simulink model "sim2"  (R2025a)
settings: Solver=VariableStepAuto  StartTime=0.0  StopTime=10.0  RelTol=1e-3
values from neighbouring files (symbols this model uses):
  D = 0.25    [lw6.m]
  i_p = n_nom/n_rpm    (= 14.0622222222)    [lw6.m]
  J_gv = ro_gv*pi*(D/2)^4*h/2    (= 0.0118116520667)    [lw6.m]
  J_sum = 35.9e-7    (= 3.59e-06)    [lw6.m]
  k1 = 0.194    [lw6.m]
  k2 = 0.032    [lw6.m]
  k_m = 19.9e-3    (= 0.0199)    [lw6.m]
  L_a = 0.070e-3    (= 7e-05)    [lw6.m]
  Lxb = 0.19    [lw7.m]
  Lym = 0.31    [lw7.m]
  Lzb = 0.21    [lw7.m]
  R_a = 0.358    [lw6.m]
  ro = 1000    [lw6.m]
  Sat_low = -20    [lw7.m]
  Sat_up = 20    [lw7.m]
  U_nom = 18    [lw6.m]
  w_0 = n_0 * 2 * pi / 60    (= 899.542696478)    [lw6.m]
settings Model: Creator=user  LastModifiedBy=user

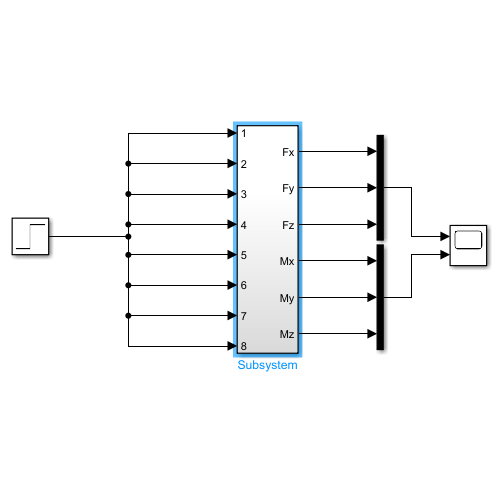
[thumbnail: Simulink's stored preview of the top-level diagram]
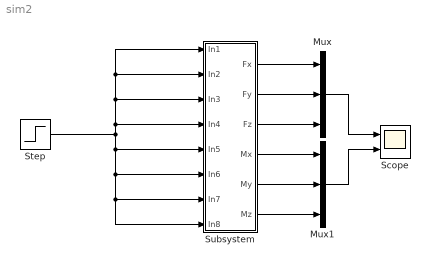
== system sim2 ==
  Mux : Mux  Inputs=3
  Mux1 : Mux  Inputs=3
  Scope : Scope  NumInputPorts=2
  Step : Step  SampleTime=0
  Subsystem : Subsystem
  wires:
  Step/1 -> Subsystem/7(In7), Subsystem/8(In8), Subsystem/6(In6), Subsystem/5(In5), Subsystem/3(In3), Subsystem/2(In2), Subsystem/1(In1), Subsystem/4(In4)
  Subsystem/1(Fx) -> Mux/1
  Subsystem/2(Fy) -> Mux/2
  Subsystem/3(Fz) -> Mux/3
  Subsystem/4(Mx) -> Mux1/1
  Subsystem/5(My) -> Mux1/2
  Subsystem/6(Mz) -> Mux1/3
  Mux/1 -> Scope/1
  Mux1/1 -> Scope/2

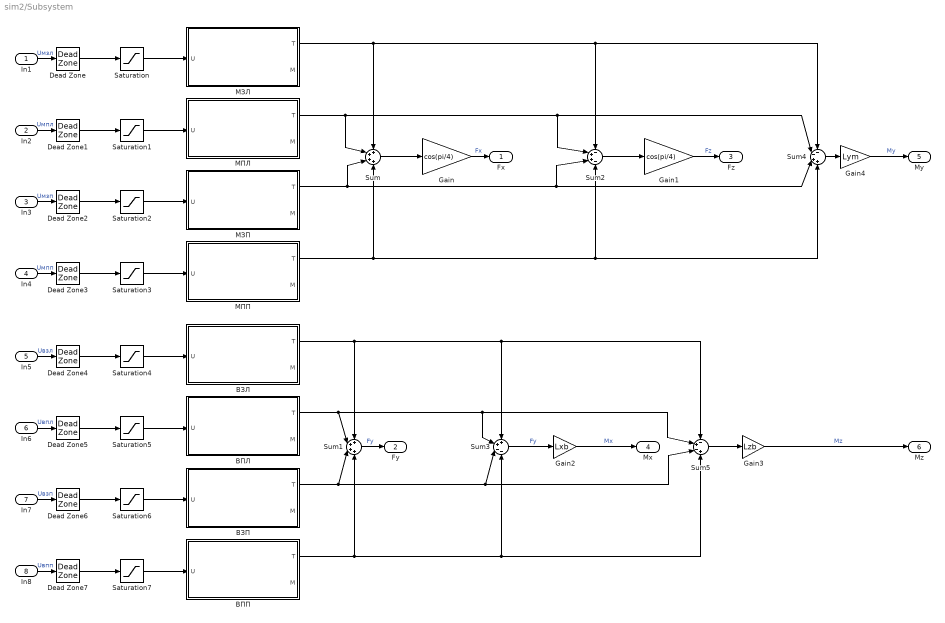
== system sim2/Subsystem ==
  In1 : Inport
  In2 : Inport  Port=2
  In3 : Inport  Port=3
  In4 : Inport  Port=4
  In5 : Inport  Port=5
  In6 : Inport  Port=6
  In7 : Inport  Port=7
  In8 : Inport  Port=8
  Dead Zone{,1..7} (8 alike) : DeadZone  LowerValue=Dead_low  UpperValue=Dead_up
  Gain : Gain  Gain=cos(pi/4)
  Gain1 : Gain  Gain=cos(pi/4)
  Gain2 : Gain  Gain=Lxb
  Gain3 : Gain  Gain=Lzb
  Gain4 : Gain  Gain=Lym
  Saturation{,1..7} (8 alike) : Saturate  UpperLimit=Sat_up  LowerLimit=Sat_low
  Sum : Sum  Inputs=++++
  Sum1 : Sum  Inputs=++++
  Sum2 : Sum  Inputs=-++-
  Sum3 : Sum  Inputs=++--
  Sum4 : Sum  Inputs=--++
  Sum5 : Sum  Inputs=-+-+
  ВЗЛ : Subsystem
  ВЗП : Subsystem
  ВПЛ : Subsystem
  ВПП : Subsystem
  МЗЛ : Subsystem
  МЗП : Subsystem
  МПЛ : Subsystem
  МПП : Subsystem
  Fx : Outport
  Fy : Outport  Port=2
  Fz : Outport  Port=3
  Mx : Outport  Port=4
  My : Outport  Port=5
  Mz : Outport  Port=6
  wires:
  In5/1 -> Dead Zone4/1  "Uвзл"
  Sum4/1 -> Gain4/1
  Gain1/1 -> Fz/1  "Fz"
  Sum5/1 -> Gain3/1
  In6/1 -> Dead Zone5/1  "Uвпл"
  Gain/1 -> Fx/1  "Fx"
  Sum/1 -> Gain/1
  Sum1/1 -> Fy/1  "Fy"
  Gain4/1 -> My/1  "My"
  ВЗП/1(T) -> Sum5/3, Sum3/3, Sum1/3
  In4/1 -> Dead Zone3/1  "Uмпп"
  Sum3/1 -> Gain2/1  "Fy"
  In8/1 -> Dead Zone7/1  "Uвпп"
  Sum2/1 -> Gain1/1
  МЗЛ/1(T) -> Sum4/1, Sum2/1, Sum/1
  ВПЛ/1(T) -> Sum5/2, Sum3/2, Sum1/2
  In2/1 -> Dead Zone1/1  "Uмпл"
  In1/1 -> Dead Zone/1  "Uмзл"
  In7/1 -> Dead Zone6/1  "Uвзп"
  Dead Zone3/1 -> Saturation3/1
  МЗП/1(T) -> Sum4/3, Sum2/3, Sum/3
  МПЛ/1(T) -> Sum4/2, Sum2/2, Sum/2
  МПП/1(T) -> Sum4/4, Sum2/4, Sum/4
  Saturation7/1 -> ВПП/1(U)
  Saturation3/1 -> МПП/1(U)
  Saturation6/1 -> ВЗП/1(U)
  Saturation2/1 -> МЗП/1(U)
  Dead Zone1/1 -> Saturation1/1
  Dead Zone2/1 -> Saturation2/1
  In3/1 -> Dead Zone2/1  "Uмзп"
  ВПП/1(T) -> Sum5/4, Sum3/4, Sum1/4
  Saturation/1 -> МЗЛ/1(U)
  Gain3/1 -> Mz/1  "Mz"
  Saturation5/1 -> ВПЛ/1(U)
  ВЗЛ/1(T) -> Sum5/1, Sum3/1, Sum1/1
  Dead Zone7/1 -> Saturation7/1
  Dead Zone4/1 -> Saturation4/1
  Gain2/1 -> Mx/1  "Mx"
  Dead Zone5/1 -> Saturation5/1
  Dead Zone/1 -> Saturation/1
  Dead Zone6/1 -> Saturation6/1
  Saturation4/1 -> ВЗЛ/1(U)
  Saturation1/1 -> МПЛ/1(U)

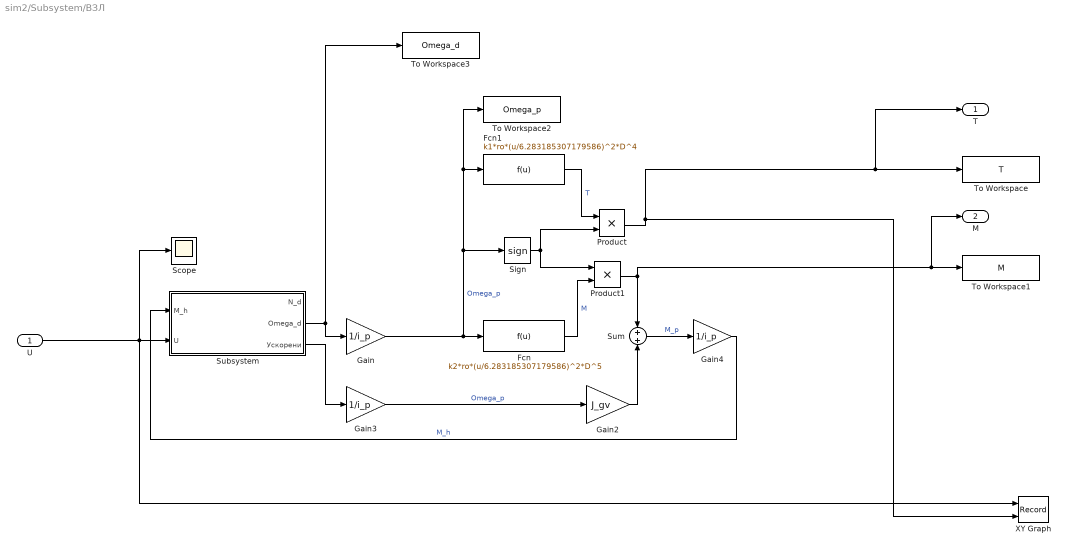
== system sim2/Subsystem/ВЗЛ ==
  U : Inport
  Fcn : Fcn  Expr=k2*ro*(u/6.283185307179586)^2*D^5
  Fcn1 : Fcn  Expr=k1*ro*(u/6.283185307179586)^2*D^4
  Gain : Gain  Gain=1/i_p
  Gain2 : Gain  Gain=J_gv
  Gain3 : Gain  Gain=1/i_p
  Gain4 : Gain  Gain=1/i_p
  Product : Product
  Product1 : Product
  Scope : Scope
      settings: ActiveDisplayYMinimum=-1  ActiveDisplayYMaximum=1
  Sign : Signum
  Subsystem : Subsystem
  Sum : Sum
  To Workspace : ToWorkspace  VariableName=T  SaveFormat=Timeseries  SampleTime=-1
  To Workspace1 : ToWorkspace  VariableName=M  SaveFormat=Timeseries  SampleTime=-1
  To Workspace2 : ToWorkspace  VariableName=Omega_p  SaveFormat=Timeseries  SampleTime=-1
  To Workspace3 : ToWorkspace  VariableName=Omega_d  SaveFormat=Timeseries  SampleTime=-1
  XY Graph : Record  NumPorts=2.0  FileSettingsInternal="{\"entries\":[{\"content\":{\"excelSettings\":{\"content\":{},\"type\":\"Streamout.ExcelSettings\"},\"parquetSettings\":{\"content\":{},\"type\":\"Streamout.ParquetSettings\"}},\"type\":\"Streamout.FileSettingStorage\",\"uuid\":\"\"}],\"packageUris\":[\"http:\\/\\/schema.mathworks.com\\/mf0\\/streamout_blocks\\/R2020a\"],\"version\":\"1.0\"}"  FrameSettings=[0, 0]  Layout=[1 1]  SignalsInternal="{\"entries\":[{\"content\":{\"signals\":[{\"content\":{\"blockPath\":[],\"dimensions\":[1],\"domain\":\"\",\"lineColor\":\"#a2142f\",\"plots\":[ 1 ],\"port\":1,\"signalID\":1,\"signalName\":\"Manual Switch\"},\"type\":\"RecordBlkView.Signal\",\"uuid\":\"\"},{\"content\":{\"blockPath\":[],\"dimensions\":[1],\"domain\":\"\",\"lineColor\":\"#139fff\",\"plots\":[ 1 ],\"port\":2,\"signalID\":2,\"signalName\":\"Product\"},\"type\":\"RecordBlkView.Signal\",\"uuid\":\"\"}]},\"type\":\"RecordBlkView.InputSignals\",\"uuid\":\"\"}],\"packageUris\":[\"http:\\/\\/schema.mathworks.com\\/mf0\\/streamout_blocks\\/R2020a\"],\"version\":\"1.0\"}"  VisualizationBindings="{\"xyplotplugin\":{\"info\":[{\"series\":[{\"bindingParametersList\":[{\"parameter\":\"X-Axis\",\"signalID\":1,\"signalName\":\"Manual Switch\"},{\"parameter\":\"Y-Axis\",\"signalID\":2,\"signalName\":\"Product\"}],\"seriesID\":0}],\"subplotID\":1}]}}"  CompatibilityTag=XY
  T : Outport
  M : Outport  Port=2
  wires:
  Gain3/1 -> Gain2/1  "Omega_p"
  Subsystem/3(Ускорени) -> Gain3/1
  Fcn1/1 -> Product/1  "T"
  Subsystem/2(Omega_d) -> Gain/1, To Workspace3/1
  Gain/1 -> Fcn/1, To Workspace2/1, Fcn1/1, Sign/1  "Omega_p"
  Sum/1 -> Gain4/1  "M_p"
  Sign/1 -> Product/2, Product1/1
  Product/1 -> T/1, To Workspace/1, XY Graph/2
  Gain4/1 -> Subsystem/1(M_h)  "M_h"
  Product1/1 -> Sum/1, M/1, To Workspace1/1
  U/1 -> Scope/1, XY Graph/1, Subsystem/2(U)
  Fcn/1 -> Product1/2  "M"
  Gain2/1 -> Sum/2

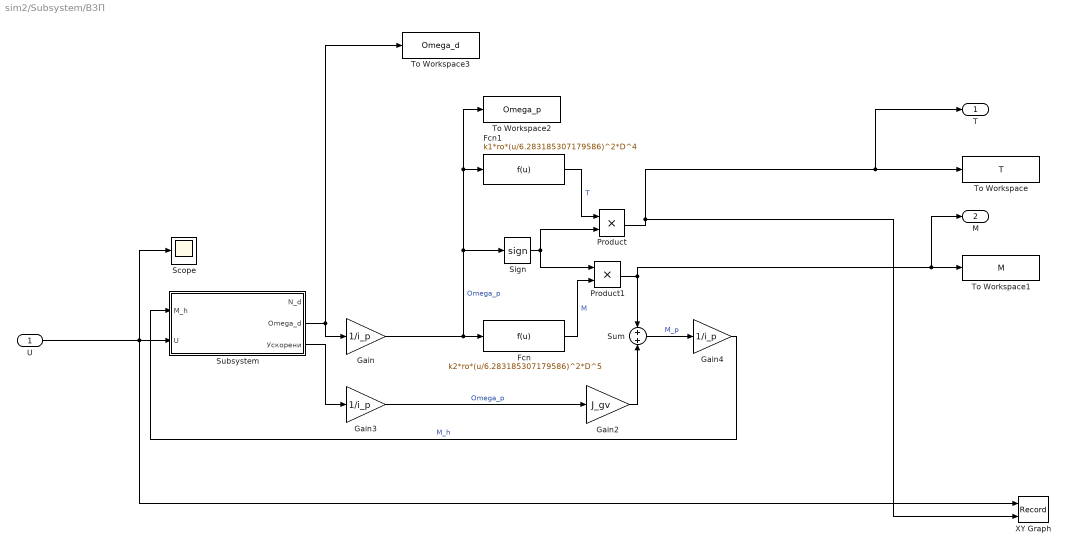
== system sim2/Subsystem/ВЗП ==
  U : Inport
  Fcn : Fcn  Expr=k2*ro*(u/6.283185307179586)^2*D^5
  Fcn1 : Fcn  Expr=k1*ro*(u/6.283185307179586)^2*D^4
  Gain : Gain  Gain=1/i_p
  Gain2 : Gain  Gain=J_gv
  Gain3 : Gain  Gain=1/i_p
  Gain4 : Gain  Gain=1/i_p
  Product : Product
  Product1 : Product
  Scope : Scope
      settings: ActiveDisplayYMinimum=-1  ActiveDisplayYMaximum=1
  Sign : Signum
  Subsystem : Subsystem
  Sum : Sum
  To Workspace : ToWorkspace  VariableName=T  SaveFormat=Timeseries  SampleTime=-1
  To Workspace1 : ToWorkspace  VariableName=M  SaveFormat=Timeseries  SampleTime=-1
  To Workspace2 : ToWorkspace  VariableName=Omega_p  SaveFormat=Timeseries  SampleTime=-1
  To Workspace3 : ToWorkspace  VariableName=Omega_d  SaveFormat=Timeseries  SampleTime=-1
  XY Graph : Record  NumPorts=2.0  FileSettingsInternal="{\"entries\":[{\"content\":{\"excelSettings\":{\"content\":{},\"type\":\"Streamout.ExcelSettings\"},\"parquetSettings\":{\"content\":{},\"type\":\"Streamout.ParquetSettings\"}},\"type\":\"Streamout.FileSettingStorage\",\"uuid\":\"\"}],\"packageUris\":[\"http:\\/\\/schema.mathworks.com\\/mf0\\/streamout_blocks\\/R2020a\"],\"version\":\"1.0\"}"  FrameSettings=[0, 0]  Layout=[1 1]  SignalsInternal="{\"entries\":[{\"content\":{\"signals\":[{\"content\":{\"blockPath\":[],\"dimensions\":[1],\"domain\":\"\",\"lineColor\":\"#a2142f\",\"plots\":[ 1 ],\"port\":1,\"signalID\":1,\"signalName\":\"Manual Switch\"},\"type\":\"RecordBlkView.Signal\",\"uuid\":\"\"},{\"content\":{\"blockPath\":[],\"dimensions\":[1],\"domain\":\"\",\"lineColor\":\"#139fff\",\"plots\":[ 1 ],\"port\":2,\"signalID\":2,\"signalName\":\"Product\"},\"type\":\"RecordBlkView.Signal\",\"uuid\":\"\"}]},\"type\":\"RecordBlkView.InputSignals\",\"uuid\":\"\"}],\"packageUris\":[\"http:\\/\\/schema.mathworks.com\\/mf0\\/streamout_blocks\\/R2020a\"],\"version\":\"1.0\"}"  VisualizationBindings="{\"xyplotplugin\":{\"info\":[{\"series\":[{\"bindingParametersList\":[{\"parameter\":\"X-Axis\",\"signalID\":1,\"signalName\":\"Manual Switch\"},{\"parameter\":\"Y-Axis\",\"signalID\":2,\"signalName\":\"Product\"}],\"seriesID\":0}],\"subplotID\":1}]}}"  CompatibilityTag=XY
  T : Outport
  M : Outport  Port=2
  wires:
  Gain3/1 -> Gain2/1  "Omega_p"
  Subsystem/3(Ускорени) -> Gain3/1
  Fcn1/1 -> Product/1  "T"
  Subsystem/2(Omega_d) -> Gain/1, To Workspace3/1
  Gain/1 -> Fcn/1, To Workspace2/1, Fcn1/1, Sign/1  "Omega_p"
  Sum/1 -> Gain4/1  "M_p"
  Sign/1 -> Product/2, Product1/1
  Product/1 -> T/1, To Workspace/1, XY Graph/2
  Gain4/1 -> Subsystem/1(M_h)  "M_h"
  Product1/1 -> Sum/1, M/1, To Workspace1/1
  U/1 -> Scope/1, XY Graph/1, Subsystem/2(U)
  Fcn/1 -> Product1/2  "M"
  Gain2/1 -> Sum/2

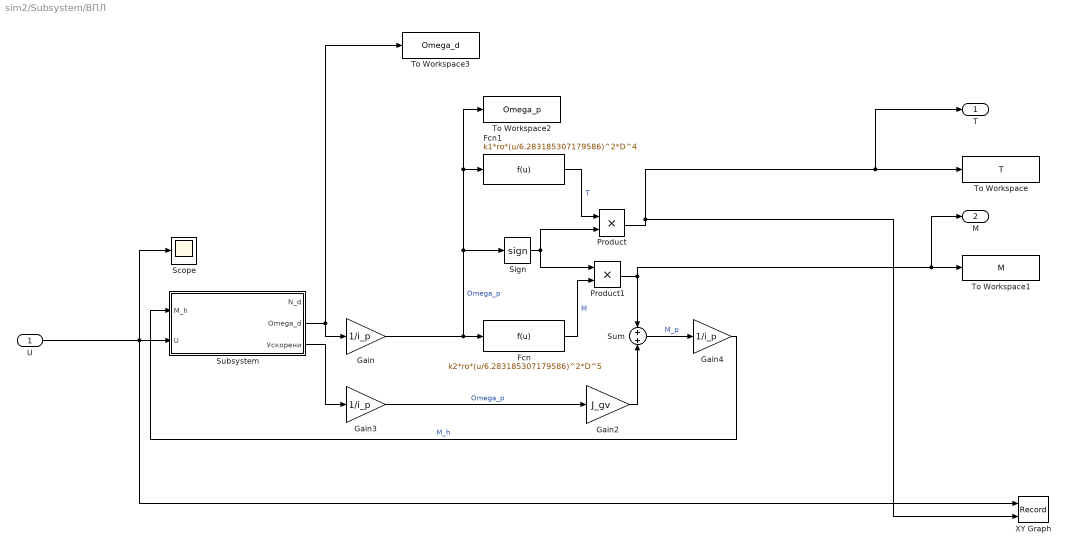
== system sim2/Subsystem/ВПЛ ==
  U : Inport
  Fcn : Fcn  Expr=k2*ro*(u/6.283185307179586)^2*D^5
  Fcn1 : Fcn  Expr=k1*ro*(u/6.283185307179586)^2*D^4
  Gain : Gain  Gain=1/i_p
  Gain2 : Gain  Gain=J_gv
  Gain3 : Gain  Gain=1/i_p
  Gain4 : Gain  Gain=1/i_p
  Product : Product
  Product1 : Product
  Scope : Scope
      settings: ActiveDisplayYMinimum=-1  ActiveDisplayYMaximum=1
  Sign : Signum
  Subsystem : Subsystem
  Sum : Sum
  To Workspace : ToWorkspace  VariableName=T  SaveFormat=Timeseries  SampleTime=-1
  To Workspace1 : ToWorkspace  VariableName=M  SaveFormat=Timeseries  SampleTime=-1
  To Workspace2 : ToWorkspace  VariableName=Omega_p  SaveFormat=Timeseries  SampleTime=-1
  To Workspace3 : ToWorkspace  VariableName=Omega_d  SaveFormat=Timeseries  SampleTime=-1
  XY Graph : Record  NumPorts=2.0  FileSettingsInternal="{\"entries\":[{\"content\":{\"excelSettings\":{\"content\":{},\"type\":\"Streamout.ExcelSettings\"},\"parquetSettings\":{\"content\":{},\"type\":\"Streamout.ParquetSettings\"}},\"type\":\"Streamout.FileSettingStorage\",\"uuid\":\"\"}],\"packageUris\":[\"http:\\/\\/schema.mathworks.com\\/mf0\\/streamout_blocks\\/R2020a\"],\"version\":\"1.0\"}"  FrameSettings=[0, 0]  Layout=[1 1]  SignalsInternal="{\"entries\":[{\"content\":{\"signals\":[{\"content\":{\"blockPath\":[],\"dimensions\":[1],\"domain\":\"\",\"lineColor\":\"#a2142f\",\"plots\":[ 1 ],\"port\":1,\"signalID\":1,\"signalName\":\"Manual Switch\"},\"type\":\"RecordBlkView.Signal\",\"uuid\":\"\"},{\"content\":{\"blockPath\":[],\"dimensions\":[1],\"domain\":\"\",\"lineColor\":\"#139fff\",\"plots\":[ 1 ],\"port\":2,\"signalID\":2,\"signalName\":\"Product\"},\"type\":\"RecordBlkView.Signal\",\"uuid\":\"\"}]},\"type\":\"RecordBlkView.InputSignals\",\"uuid\":\"\"}],\"packageUris\":[\"http:\\/\\/schema.mathworks.com\\/mf0\\/streamout_blocks\\/R2020a\"],\"version\":\"1.0\"}"  VisualizationBindings="{\"xyplotplugin\":{\"info\":[{\"series\":[{\"bindingParametersList\":[{\"parameter\":\"X-Axis\",\"signalID\":1,\"signalName\":\"Manual Switch\"},{\"parameter\":\"Y-Axis\",\"signalID\":2,\"signalName\":\"Product\"}],\"seriesID\":0}],\"subplotID\":1}]}}"  CompatibilityTag=XY
  T : Outport
  M : Outport  Port=2
  wires:
  Gain3/1 -> Gain2/1  "Omega_p"
  Subsystem/3(Ускорени) -> Gain3/1
  Fcn1/1 -> Product/1  "T"
  Subsystem/2(Omega_d) -> Gain/1, To Workspace3/1
  Gain/1 -> Fcn/1, To Workspace2/1, Fcn1/1, Sign/1  "Omega_p"
  Sum/1 -> Gain4/1  "M_p"
  Sign/1 -> Product/2, Product1/1
  Product/1 -> T/1, To Workspace/1, XY Graph/2
  Gain4/1 -> Subsystem/1(M_h)  "M_h"
  Product1/1 -> Sum/1, M/1, To Workspace1/1
  U/1 -> Scope/1, XY Graph/1, Subsystem/2(U)
  Fcn/1 -> Product1/2  "M"
  Gain2/1 -> Sum/2

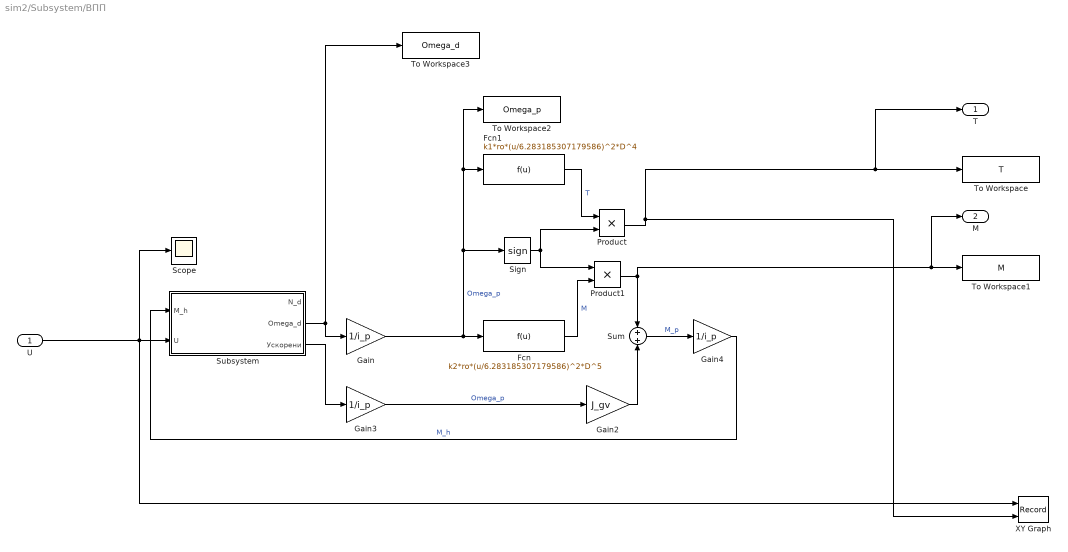
== system sim2/Subsystem/ВПП ==
  U : Inport
  Fcn : Fcn  Expr=k2*ro*(u/6.283185307179586)^2*D^5
  Fcn1 : Fcn  Expr=k1*ro*(u/6.283185307179586)^2*D^4
  Gain : Gain  Gain=1/i_p
  Gain2 : Gain  Gain=J_gv
  Gain3 : Gain  Gain=1/i_p
  Gain4 : Gain  Gain=1/i_p
  Product : Product
  Product1 : Product
  Scope : Scope
      settings: ActiveDisplayYMinimum=-1  ActiveDisplayYMaximum=1
  Sign : Signum
  Subsystem : Subsystem
  Sum : Sum
  To Workspace : ToWorkspace  VariableName=T  SaveFormat=Timeseries  SampleTime=-1
  To Workspace1 : ToWorkspace  VariableName=M  SaveFormat=Timeseries  SampleTime=-1
  To Workspace2 : ToWorkspace  VariableName=Omega_p  SaveFormat=Timeseries  SampleTime=-1
  To Workspace3 : ToWorkspace  VariableName=Omega_d  SaveFormat=Timeseries  SampleTime=-1
  XY Graph : Record  NumPorts=2.0  FileSettingsInternal="{\"entries\":[{\"content\":{\"excelSettings\":{\"content\":{},\"type\":\"Streamout.ExcelSettings\"},\"parquetSettings\":{\"content\":{},\"type\":\"Streamout.ParquetSettings\"}},\"type\":\"Streamout.FileSettingStorage\",\"uuid\":\"\"}],\"packageUris\":[\"http:\\/\\/schema.mathworks.com\\/mf0\\/streamout_blocks\\/R2020a\"],\"version\":\"1.0\"}"  FrameSettings=[0, 0]  Layout=[1 1]  SignalsInternal="{\"entries\":[{\"content\":{\"signals\":[{\"content\":{\"blockPath\":[],\"dimensions\":[1],\"domain\":\"\",\"lineColor\":\"#a2142f\",\"plots\":[ 1 ],\"port\":1,\"signalID\":1,\"signalName\":\"Manual Switch\"},\"type\":\"RecordBlkView.Signal\",\"uuid\":\"\"},{\"content\":{\"blockPath\":[],\"dimensions\":[1],\"domain\":\"\",\"lineColor\":\"#139fff\",\"plots\":[ 1 ],\"port\":2,\"signalID\":2,\"signalName\":\"Product\"},\"type\":\"RecordBlkView.Signal\",\"uuid\":\"\"}]},\"type\":\"RecordBlkView.InputSignals\",\"uuid\":\"\"}],\"packageUris\":[\"http:\\/\\/schema.mathworks.com\\/mf0\\/streamout_blocks\\/R2020a\"],\"version\":\"1.0\"}"  VisualizationBindings="{\"xyplotplugin\":{\"info\":[{\"series\":[{\"bindingParametersList\":[{\"parameter\":\"X-Axis\",\"signalID\":1,\"signalName\":\"Manual Switch\"},{\"parameter\":\"Y-Axis\",\"signalID\":2,\"signalName\":\"Product\"}],\"seriesID\":0}],\"subplotID\":1}]}}"  CompatibilityTag=XY
  T : Outport
  M : Outport  Port=2
  wires:
  Gain3/1 -> Gain2/1  "Omega_p"
  Subsystem/3(Ускорени) -> Gain3/1
  Fcn1/1 -> Product/1  "T"
  Subsystem/2(Omega_d) -> Gain/1, To Workspace3/1
  Gain/1 -> Fcn/1, To Workspace2/1, Fcn1/1, Sign/1  "Omega_p"
  Sum/1 -> Gain4/1  "M_p"
  Sign/1 -> Product/2, Product1/1
  Product/1 -> T/1, To Workspace/1, XY Graph/2
  Gain4/1 -> Subsystem/1(M_h)  "M_h"
  Product1/1 -> Sum/1, M/1, To Workspace1/1
  U/1 -> Scope/1, XY Graph/1, Subsystem/2(U)
  Fcn/1 -> Product1/2  "M"
  Gain2/1 -> Sum/2

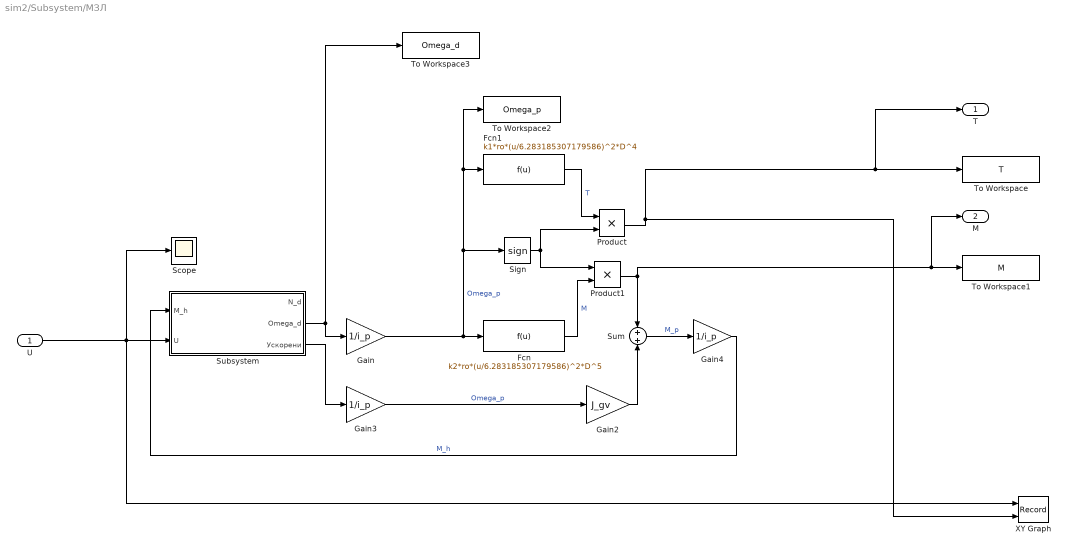
== system sim2/Subsystem/МЗЛ ==
  U : Inport
  Fcn : Fcn  Expr=k2*ro*(u/6.283185307179586)^2*D^5
  Fcn1 : Fcn  Expr=k1*ro*(u/6.283185307179586)^2*D^4
  Gain : Gain  Gain=1/i_p
  Gain2 : Gain  Gain=J_gv
  Gain3 : Gain  Gain=1/i_p
  Gain4 : Gain  Gain=1/i_p
  Product : Product
  Product1 : Product
  Scope : Scope
      settings: ActiveDisplayYMinimum=-1  ActiveDisplayYMaximum=1
  Sign : Signum
  Subsystem : Subsystem
  Sum : Sum
  To Workspace : ToWorkspace  VariableName=T  SaveFormat=Timeseries  SampleTime=-1
  To Workspace1 : ToWorkspace  VariableName=M  SaveFormat=Timeseries  SampleTime=-1
  To Workspace2 : ToWorkspace  VariableName=Omega_p  SaveFormat=Timeseries  SampleTime=-1
  To Workspace3 : ToWorkspace  VariableName=Omega_d  SaveFormat=Timeseries  SampleTime=-1
  XY Graph : Record  NumPorts=2.0  FileSettingsInternal="{\"entries\":[{\"content\":{\"excelSettings\":{\"content\":{},\"type\":\"Streamout.ExcelSettings\"},\"parquetSettings\":{\"content\":{},\"type\":\"Streamout.ParquetSettings\"}},\"type\":\"Streamout.FileSettingStorage\",\"uuid\":\"\"}],\"packageUris\":[\"http:\\/\\/schema.mathworks.com\\/mf0\\/streamout_blocks\\/R2020a\"],\"version\":\"1.0\"}"  FrameSettings=[0, 0]  Layout=[1 1]  SignalsInternal="{\"entries\":[{\"content\":{\"signals\":[{\"content\":{\"blockPath\":[],\"dimensions\":[1],\"domain\":\"\",\"lineColor\":\"#a2142f\",\"plots\":[ 1 ],\"port\":1,\"signalID\":1,\"signalName\":\"Manual Switch\"},\"type\":\"RecordBlkView.Signal\",\"uuid\":\"\"},{\"content\":{\"blockPath\":[],\"dimensions\":[1],\"domain\":\"\",\"lineColor\":\"#139fff\",\"plots\":[ 1 ],\"port\":2,\"signalID\":2,\"signalName\":\"Product\"},\"type\":\"RecordBlkView.Signal\",\"uuid\":\"\"}]},\"type\":\"RecordBlkView.InputSignals\",\"uuid\":\"\"}],\"packageUris\":[\"http:\\/\\/schema.mathworks.com\\/mf0\\/streamout_blocks\\/R2020a\"],\"version\":\"1.0\"}"  VisualizationBindings="{\"xyplotplugin\":{\"info\":[{\"series\":[{\"bindingParametersList\":[{\"parameter\":\"X-Axis\",\"signalID\":1,\"signalName\":\"Manual Switch\"},{\"parameter\":\"Y-Axis\",\"signalID\":2,\"signalName\":\"Product\"}],\"seriesID\":0}],\"subplotID\":1}]}}"  CompatibilityTag=XY
  T : Outport
  M : Outport  Port=2
  wires:
  Gain3/1 -> Gain2/1  "Omega_p"
  Subsystem/3(Ускорени) -> Gain3/1
  Fcn1/1 -> Product/1  "T"
  Subsystem/2(Omega_d) -> Gain/1, To Workspace3/1
  Gain/1 -> Fcn/1, To Workspace2/1, Fcn1/1, Sign/1  "Omega_p"
  Sum/1 -> Gain4/1  "M_p"
  Sign/1 -> Product/2, Product1/1
  Product/1 -> T/1, To Workspace/1, XY Graph/2
  Gain4/1 -> Subsystem/1(M_h)  "M_h"
  Product1/1 -> Sum/1, M/1, To Workspace1/1
  U/1 -> Subsystem/2(U), XY Graph/1, Scope/1
  Fcn/1 -> Product1/2  "M"
  Gain2/1 -> Sum/2

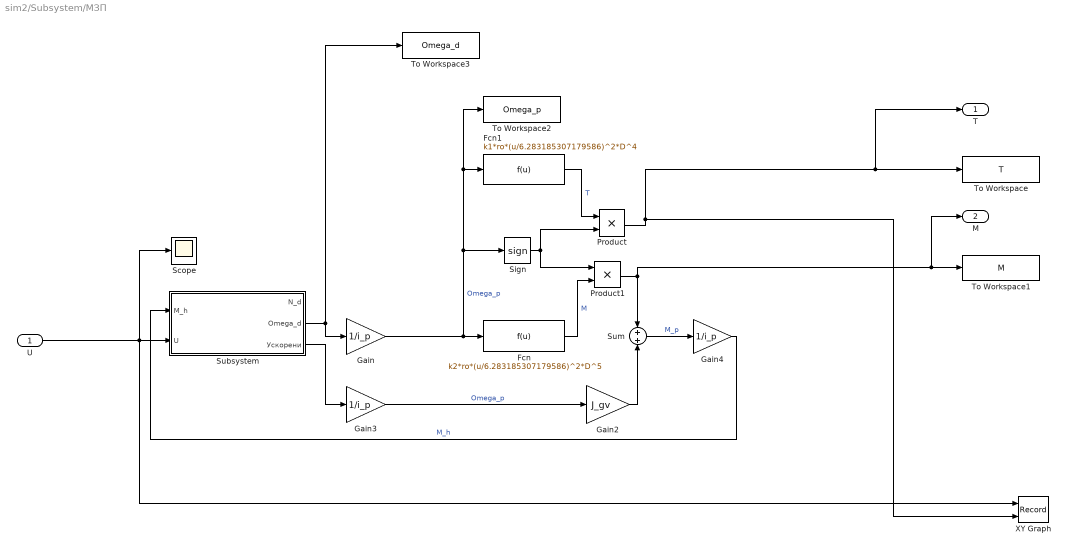
== system sim2/Subsystem/МЗП ==
  U : Inport
  Fcn : Fcn  Expr=k2*ro*(u/6.283185307179586)^2*D^5
  Fcn1 : Fcn  Expr=k1*ro*(u/6.283185307179586)^2*D^4
  Gain : Gain  Gain=1/i_p
  Gain2 : Gain  Gain=J_gv
  Gain3 : Gain  Gain=1/i_p
  Gain4 : Gain  Gain=1/i_p
  Product : Product
  Product1 : Product
  Scope : Scope
      settings: ActiveDisplayYMinimum=-1  ActiveDisplayYMaximum=1
  Sign : Signum
  Subsystem : Subsystem
  Sum : Sum
  To Workspace : ToWorkspace  VariableName=T  SaveFormat=Timeseries  SampleTime=-1
  To Workspace1 : ToWorkspace  VariableName=M  SaveFormat=Timeseries  SampleTime=-1
  To Workspace2 : ToWorkspace  VariableName=Omega_p  SaveFormat=Timeseries  SampleTime=-1
  To Workspace3 : ToWorkspace  VariableName=Omega_d  SaveFormat=Timeseries  SampleTime=-1
  XY Graph : Record  NumPorts=2.0  FileSettingsInternal="{\"entries\":[{\"content\":{\"excelSettings\":{\"content\":{},\"type\":\"Streamout.ExcelSettings\"},\"parquetSettings\":{\"content\":{},\"type\":\"Streamout.ParquetSettings\"}},\"type\":\"Streamout.FileSettingStorage\",\"uuid\":\"\"}],\"packageUris\":[\"http:\\/\\/schema.mathworks.com\\/mf0\\/streamout_blocks\\/R2020a\"],\"version\":\"1.0\"}"  FrameSettings=[0, 0]  Layout=[1 1]  SignalsInternal="{\"entries\":[{\"content\":{\"signals\":[{\"content\":{\"blockPath\":[],\"dimensions\":[1],\"domain\":\"\",\"lineColor\":\"#a2142f\",\"plots\":[ 1 ],\"port\":1,\"signalID\":1,\"signalName\":\"Manual Switch\"},\"type\":\"RecordBlkView.Signal\",\"uuid\":\"\"},{\"content\":{\"blockPath\":[],\"dimensions\":[1],\"domain\":\"\",\"lineColor\":\"#139fff\",\"plots\":[ 1 ],\"port\":2,\"signalID\":2,\"signalName\":\"Product\"},\"type\":\"RecordBlkView.Signal\",\"uuid\":\"\"}]},\"type\":\"RecordBlkView.InputSignals\",\"uuid\":\"\"}],\"packageUris\":[\"http:\\/\\/schema.mathworks.com\\/mf0\\/streamout_blocks\\/R2020a\"],\"version\":\"1.0\"}"  VisualizationBindings="{\"xyplotplugin\":{\"info\":[{\"series\":[{\"bindingParametersList\":[{\"parameter\":\"X-Axis\",\"signalID\":1,\"signalName\":\"Manual Switch\"},{\"parameter\":\"Y-Axis\",\"signalID\":2,\"signalName\":\"Product\"}],\"seriesID\":0}],\"subplotID\":1}]}}"  CompatibilityTag=XY
  T : Outport
  M : Outport  Port=2
  wires:
  Gain3/1 -> Gain2/1  "Omega_p"
  Subsystem/3(Ускорени) -> Gain3/1
  Fcn1/1 -> Product/1  "T"
  Subsystem/2(Omega_d) -> Gain/1, To Workspace3/1
  Gain/1 -> Fcn/1, To Workspace2/1, Fcn1/1, Sign/1  "Omega_p"
  Sum/1 -> Gain4/1  "M_p"
  Sign/1 -> Product/2, Product1/1
  Product/1 -> T/1, To Workspace/1, XY Graph/2
  Gain4/1 -> Subsystem/1(M_h)  "M_h"
  Product1/1 -> Sum/1, M/1, To Workspace1/1
  U/1 -> Scope/1, XY Graph/1, Subsystem/2(U)
  Fcn/1 -> Product1/2  "M"
  Gain2/1 -> Sum/2

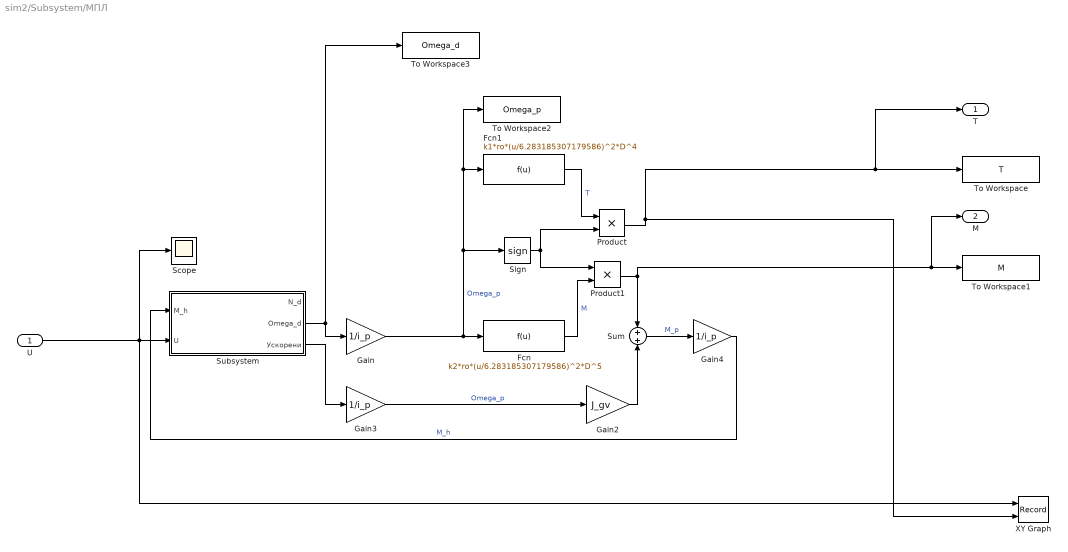
== system sim2/Subsystem/МПЛ ==
  U : Inport
  Fcn : Fcn  Expr=k2*ro*(u/6.283185307179586)^2*D^5
  Fcn1 : Fcn  Expr=k1*ro*(u/6.283185307179586)^2*D^4
  Gain : Gain  Gain=1/i_p
  Gain2 : Gain  Gain=J_gv
  Gain3 : Gain  Gain=1/i_p
  Gain4 : Gain  Gain=1/i_p
  Product : Product
  Product1 : Product
  Scope : Scope
      settings: ActiveDisplayYMinimum=-1  ActiveDisplayYMaximum=1
  Sign : Signum
  Subsystem : Subsystem
  Sum : Sum
  To Workspace : ToWorkspace  VariableName=T  SaveFormat=Timeseries  SampleTime=-1
  To Workspace1 : ToWorkspace  VariableName=M  SaveFormat=Timeseries  SampleTime=-1
  To Workspace2 : ToWorkspace  VariableName=Omega_p  SaveFormat=Timeseries  SampleTime=-1
  To Workspace3 : ToWorkspace  VariableName=Omega_d  SaveFormat=Timeseries  SampleTime=-1
  XY Graph : Record  NumPorts=2.0  FileSettingsInternal="{\"entries\":[{\"content\":{\"excelSettings\":{\"content\":{},\"type\":\"Streamout.ExcelSettings\"},\"parquetSettings\":{\"content\":{},\"type\":\"Streamout.ParquetSettings\"}},\"type\":\"Streamout.FileSettingStorage\",\"uuid\":\"\"}],\"packageUris\":[\"http:\\/\\/schema.mathworks.com\\/mf0\\/streamout_blocks\\/R2020a\"],\"version\":\"1.0\"}"  FrameSettings=[0, 0]  Layout=[1 1]  SignalsInternal="{\"entries\":[{\"content\":{\"signals\":[{\"content\":{\"blockPath\":[],\"dimensions\":[1],\"domain\":\"\",\"lineColor\":\"#a2142f\",\"plots\":[ 1 ],\"port\":1,\"signalID\":1,\"signalName\":\"Manual Switch\"},\"type\":\"RecordBlkView.Signal\",\"uuid\":\"\"},{\"content\":{\"blockPath\":[],\"dimensions\":[1],\"domain\":\"\",\"lineColor\":\"#139fff\",\"plots\":[ 1 ],\"port\":2,\"signalID\":2,\"signalName\":\"Product\"},\"type\":\"RecordBlkView.Signal\",\"uuid\":\"\"}]},\"type\":\"RecordBlkView.InputSignals\",\"uuid\":\"\"}],\"packageUris\":[\"http:\\/\\/schema.mathworks.com\\/mf0\\/streamout_blocks\\/R2020a\"],\"version\":\"1.0\"}"  VisualizationBindings="{\"xyplotplugin\":{\"info\":[{\"series\":[{\"bindingParametersList\":[{\"parameter\":\"X-Axis\",\"signalID\":1,\"signalName\":\"Manual Switch\"},{\"parameter\":\"Y-Axis\",\"signalID\":2,\"signalName\":\"Product\"}],\"seriesID\":0}],\"subplotID\":1}]}}"  CompatibilityTag=XY
  T : Outport
  M : Outport  Port=2
  wires:
  Gain3/1 -> Gain2/1  "Omega_p"
  Subsystem/3(Ускорени) -> Gain3/1
  Fcn1/1 -> Product/1  "T"
  Subsystem/2(Omega_d) -> Gain/1, To Workspace3/1
  Gain/1 -> Fcn/1, To Workspace2/1, Fcn1/1, Sign/1  "Omega_p"
  Sum/1 -> Gain4/1  "M_p"
  Sign/1 -> Product/2, Product1/1
  Product/1 -> T/1, To Workspace/1, XY Graph/2
  Gain4/1 -> Subsystem/1(M_h)  "M_h"
  Product1/1 -> Sum/1, M/1, To Workspace1/1
  U/1 -> Scope/1, XY Graph/1, Subsystem/2(U)
  Fcn/1 -> Product1/2  "M"
  Gain2/1 -> Sum/2

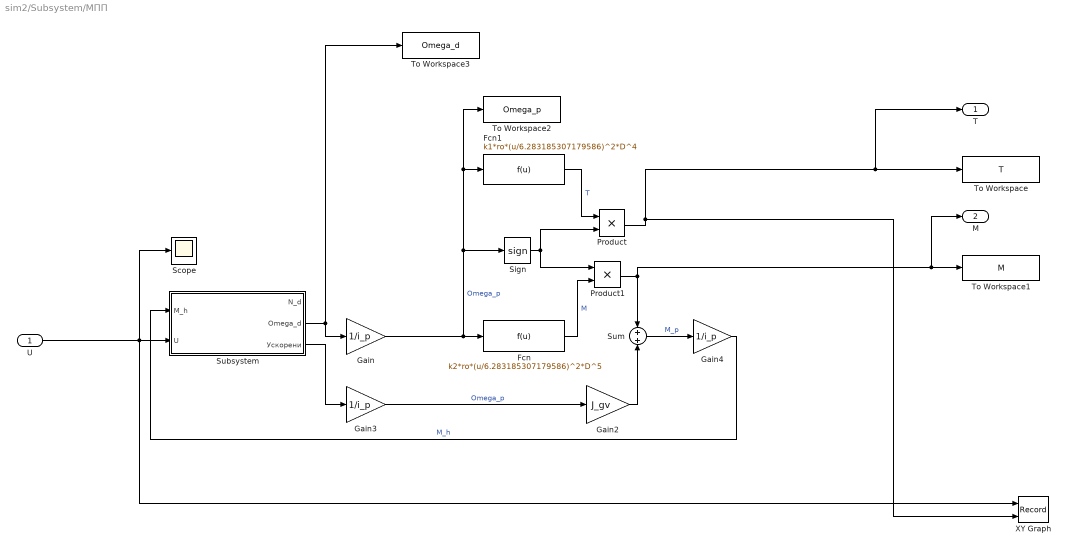
== system sim2/Subsystem/МПП ==
  U : Inport
  Fcn : Fcn  Expr=k2*ro*(u/6.283185307179586)^2*D^5
  Fcn1 : Fcn  Expr=k1*ro*(u/6.283185307179586)^2*D^4
  Gain : Gain  Gain=1/i_p
  Gain2 : Gain  Gain=J_gv
  Gain3 : Gain  Gain=1/i_p
  Gain4 : Gain  Gain=1/i_p
  Product : Product
  Product1 : Product
  Scope : Scope
      settings: ActiveDisplayYMinimum=-1  ActiveDisplayYMaximum=1
  Sign : Signum
  Subsystem : Subsystem
  Sum : Sum
  To Workspace : ToWorkspace  VariableName=T  SaveFormat=Timeseries  SampleTime=-1
  To Workspace1 : ToWorkspace  VariableName=M  SaveFormat=Timeseries  SampleTime=-1
  To Workspace2 : ToWorkspace  VariableName=Omega_p  SaveFormat=Timeseries  SampleTime=-1
  To Workspace3 : ToWorkspace  VariableName=Omega_d  SaveFormat=Timeseries  SampleTime=-1
  XY Graph : Record  NumPorts=2.0  FileSettingsInternal="{\"entries\":[{\"content\":{\"excelSettings\":{\"content\":{},\"type\":\"Streamout.ExcelSettings\"},\"parquetSettings\":{\"content\":{},\"type\":\"Streamout.ParquetSettings\"}},\"type\":\"Streamout.FileSettingStorage\",\"uuid\":\"\"}],\"packageUris\":[\"http:\\/\\/schema.mathworks.com\\/mf0\\/streamout_blocks\\/R2020a\"],\"version\":\"1.0\"}"  FrameSettings=[0, 0]  Layout=[1 1]  SignalsInternal="{\"entries\":[{\"content\":{\"signals\":[{\"content\":{\"blockPath\":[],\"dimensions\":[1],\"domain\":\"\",\"lineColor\":\"#a2142f\",\"plots\":[ 1 ],\"port\":1,\"signalID\":1,\"signalName\":\"Manual Switch\"},\"type\":\"RecordBlkView.Signal\",\"uuid\":\"\"},{\"content\":{\"blockPath\":[],\"dimensions\":[1],\"domain\":\"\",\"lineColor\":\"#139fff\",\"plots\":[ 1 ],\"port\":2,\"signalID\":2,\"signalName\":\"Product\"},\"type\":\"RecordBlkView.Signal\",\"uuid\":\"\"}]},\"type\":\"RecordBlkView.InputSignals\",\"uuid\":\"\"}],\"packageUris\":[\"http:\\/\\/schema.mathworks.com\\/mf0\\/streamout_blocks\\/R2020a\"],\"version\":\"1.0\"}"  VisualizationBindings="{\"xyplotplugin\":{\"info\":[{\"series\":[{\"bindingParametersList\":[{\"parameter\":\"X-Axis\",\"signalID\":1,\"signalName\":\"Manual Switch\"},{\"parameter\":\"Y-Axis\",\"signalID\":2,\"signalName\":\"Product\"}],\"seriesID\":0}],\"subplotID\":1}]}}"  CompatibilityTag=XY
  T : Outport
  M : Outport  Port=2
  wires:
  Gain3/1 -> Gain2/1  "Omega_p"
  Subsystem/3(Ускорени) -> Gain3/1
  Fcn1/1 -> Product/1  "T"
  Subsystem/2(Omega_d) -> Gain/1, To Workspace3/1
  Gain/1 -> Fcn/1, To Workspace2/1, Fcn1/1, Sign/1  "Omega_p"
  Sum/1 -> Gain4/1  "M_p"
  Sign/1 -> Product/2, Product1/1
  Product/1 -> T/1, To Workspace/1, XY Graph/2
  Gain4/1 -> Subsystem/1(M_h)  "M_h"
  Product1/1 -> Sum/1, M/1, To Workspace1/1
  U/1 -> Scope/1, XY Graph/1, Subsystem/2(U)
  Fcn/1 -> Product1/2  "M"
  Gain2/1 -> Sum/2

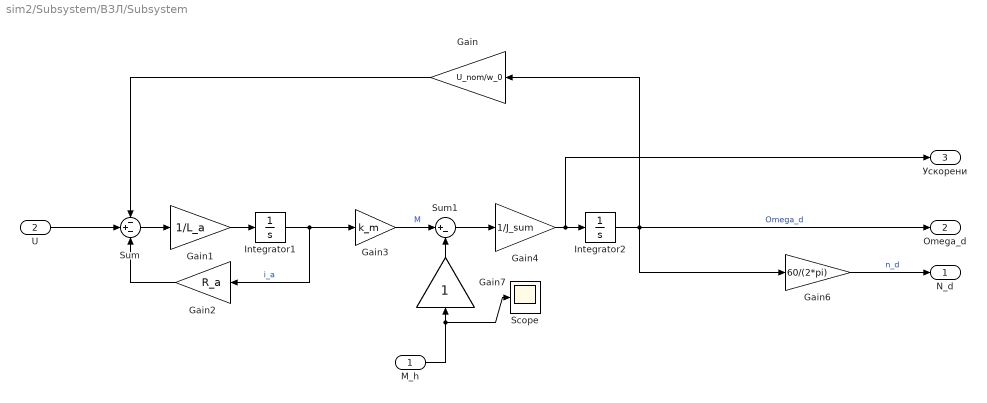
== system sim2/Subsystem/ВЗЛ/Subsystem ==
  M_h : Inport
  U : Inport  Port=2
  Gain : Gain  Gain=U_nom/w_0
  Gain1 : Gain  Gain=1/L_a
  Gain2 : Gain  Gain=R_a
  Gain3 : Gain  Gain=k_m
  Gain4 : Gain  Gain=1/J_sum
  Gain6 : Gain  Gain=60/(2*pi)
  Gain7 : Gain
  Integrator1 : Integrator
  Integrator2 : Integrator
  Scope : Scope
      settings: ActiveDisplayYMinimum=-1  ActiveDisplayYMaximum=1
  Sum : Sum  Inputs=-+-
  Sum1 : Sum  Inputs=|+-
  N_d : Outport
  Omega_d : Outport  Port=2
  Ускорени : Outport  Port=3
  wires:
  U/1 -> Sum/2
  Gain3/1 -> Sum1/1  "M"
  M_h/1 -> Scope/1, Gain7/1
  Gain6/1 -> N_d/1  "n_d"
  Gain1/1 -> Integrator1/1
  Integrator1/1 -> Gain3/1, Gain2/1  "i_a"
  Integrator2/1 -> Omega_d/1, Gain6/1, Gain/1  "Omega_d"
  Gain4/1 -> Ускорени/1, Integrator2/1
  Sum/1 -> Gain1/1
  Gain2/1 -> Sum/3
  Gain7/1 -> Sum1/2
  Gain/1 -> Sum/1
  Sum1/1 -> Gain4/1

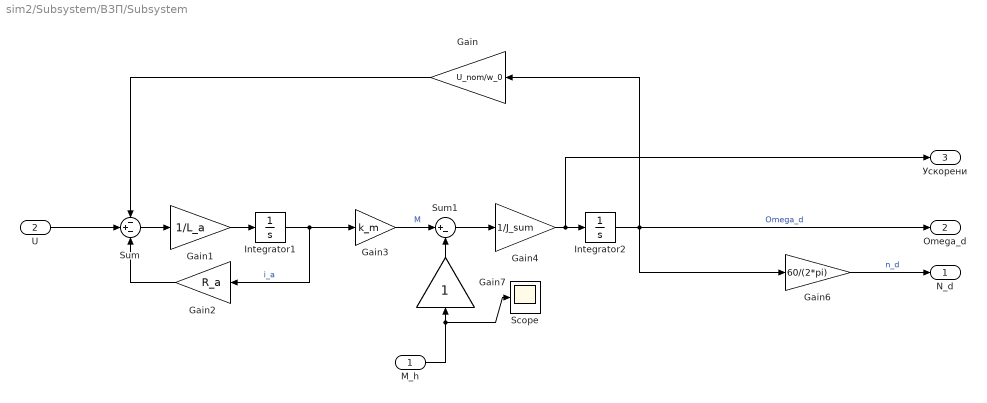
== system sim2/Subsystem/ВЗП/Subsystem ==
  M_h : Inport
  U : Inport  Port=2
  Gain : Gain  Gain=U_nom/w_0
  Gain1 : Gain  Gain=1/L_a
  Gain2 : Gain  Gain=R_a
  Gain3 : Gain  Gain=k_m
  Gain4 : Gain  Gain=1/J_sum
  Gain6 : Gain  Gain=60/(2*pi)
  Gain7 : Gain
  Integrator1 : Integrator
  Integrator2 : Integrator
  Scope : Scope
      settings: ActiveDisplayYMinimum=-1  ActiveDisplayYMaximum=1
  Sum : Sum  Inputs=-+-
  Sum1 : Sum  Inputs=|+-
  N_d : Outport
  Omega_d : Outport  Port=2
  Ускорени : Outport  Port=3
  wires:
  U/1 -> Sum/2
  Gain3/1 -> Sum1/1  "M"
  M_h/1 -> Scope/1, Gain7/1
  Gain6/1 -> N_d/1  "n_d"
  Gain1/1 -> Integrator1/1
  Integrator1/1 -> Gain3/1, Gain2/1  "i_a"
  Integrator2/1 -> Omega_d/1, Gain6/1, Gain/1  "Omega_d"
  Gain4/1 -> Ускорени/1, Integrator2/1
  Sum/1 -> Gain1/1
  Gain2/1 -> Sum/3
  Gain7/1 -> Sum1/2
  Gain/1 -> Sum/1
  Sum1/1 -> Gain4/1

== system sim2/Subsystem/ВПЛ/Subsystem ==
  M_h : Inport
  U : Inport  Port=2
  Gain : Gain  Gain=U_nom/w_0
  Gain1 : Gain  Gain=1/L_a
  Gain2 : Gain  Gain=R_a
  Gain3 : Gain  Gain=k_m
  Gain4 : Gain  Gain=1/J_sum
  Gain6 : Gain  Gain=60/(2*pi)
  Gain7 : Gain
  Integrator1 : Integrator
  Integrator2 : Integrator
  Scope : Scope
      settings: ActiveDisplayYMinimum=-1  ActiveDisplayYMaximum=1
  Sum : Sum  Inputs=-+-
  Sum1 : Sum  Inputs=|+-
  N_d : Outport
  Omega_d : Outport  Port=2
  Ускорени : Outport  Port=3
  wires:
  U/1 -> Sum/2
  Gain3/1 -> Sum1/1  "M"
  M_h/1 -> Scope/1, Gain7/1
  Gain6/1 -> N_d/1  "n_d"
  Gain1/1 -> Integrator1/1
  Integrator1/1 -> Gain3/1, Gain2/1  "i_a"
  Integrator2/1 -> Omega_d/1, Gain6/1, Gain/1  "Omega_d"
  Gain4/1 -> Ускорени/1, Integrator2/1
  Sum/1 -> Gain1/1
  Gain2/1 -> Sum/3
  Gain7/1 -> Sum1/2
  Gain/1 -> Sum/1
  Sum1/1 -> Gain4/1

== system sim2/Subsystem/ВПП/Subsystem ==
  M_h : Inport
  U : Inport  Port=2
  Gain : Gain  Gain=U_nom/w_0
  Gain1 : Gain  Gain=1/L_a
  Gain2 : Gain  Gain=R_a
  Gain3 : Gain  Gain=k_m
  Gain4 : Gain  Gain=1/J_sum
  Gain6 : Gain  Gain=60/(2*pi)
  Gain7 : Gain
  Integrator1 : Integrator
  Integrator2 : Integrator
  Scope : Scope
      settings: ActiveDisplayYMinimum=-1  ActiveDisplayYMaximum=1
  Sum : Sum  Inputs=-+-
  Sum1 : Sum  Inputs=|+-
  N_d : Outport
  Omega_d : Outport  Port=2
  Ускорени : Outport  Port=3
  wires:
  U/1 -> Sum/2
  Gain3/1 -> Sum1/1  "M"
  M_h/1 -> Scope/1, Gain7/1
  Gain6/1 -> N_d/1  "n_d"
  Gain1/1 -> Integrator1/1
  Integrator1/1 -> Gain3/1, Gain2/1  "i_a"
  Integrator2/1 -> Omega_d/1, Gain6/1, Gain/1  "Omega_d"
  Gain4/1 -> Ускорени/1, Integrator2/1
  Sum/1 -> Gain1/1
  Gain2/1 -> Sum/3
  Gain7/1 -> Sum1/2
  Gain/1 -> Sum/1
  Sum1/1 -> Gain4/1

== system sim2/Subsystem/МЗЛ/Subsystem ==
  M_h : Inport
  U : Inport  Port=2
  Gain : Gain  Gain=U_nom/w_0
  Gain1 : Gain  Gain=1/L_a
  Gain2 : Gain  Gain=R_a
  Gain3 : Gain  Gain=k_m
  Gain4 : Gain  Gain=1/J_sum
  Gain6 : Gain  Gain=60/(2*pi)
  Gain7 : Gain
  Integrator1 : Integrator
  Integrator2 : Integrator
  Scope : Scope
      settings: ActiveDisplayYMinimum=-1  ActiveDisplayYMaximum=1
  Sum : Sum  Inputs=-+-
  Sum1 : Sum  Inputs=|+-
  N_d : Outport
  Omega_d : Outport  Port=2
  Ускорени : Outport  Port=3
  wires:
  U/1 -> Sum/2
  Gain3/1 -> Sum1/1  "M"
  M_h/1 -> Scope/1, Gain7/1
  Gain6/1 -> N_d/1  "n_d"
  Gain1/1 -> Integrator1/1
  Integrator1/1 -> Gain3/1, Gain2/1  "i_a"
  Integrator2/1 -> Omega_d/1, Gain6/1, Gain/1  "Omega_d"
  Gain4/1 -> Ускорени/1, Integrator2/1
  Sum/1 -> Gain1/1
  Gain2/1 -> Sum/3
  Gain7/1 -> Sum1/2
  Gain/1 -> Sum/1
  Sum1/1 -> Gain4/1

== system sim2/Subsystem/МЗП/Subsystem ==
  M_h : Inport
  U : Inport  Port=2
  Gain : Gain  Gain=U_nom/w_0
  Gain1 : Gain  Gain=1/L_a
  Gain2 : Gain  Gain=R_a
  Gain3 : Gain  Gain=k_m
  Gain4 : Gain  Gain=1/J_sum
  Gain6 : Gain  Gain=60/(2*pi)
  Gain7 : Gain
  Integrator1 : Integrator
  Integrator2 : Integrator
  Scope : Scope
      settings: ActiveDisplayYMinimum=-1  ActiveDisplayYMaximum=1
  Sum : Sum  Inputs=-+-
  Sum1 : Sum  Inputs=|+-
  N_d : Outport
  Omega_d : Outport  Port=2
  Ускорени : Outport  Port=3
  wires:
  U/1 -> Sum/2
  Gain3/1 -> Sum1/1  "M"
  M_h/1 -> Scope/1, Gain7/1
  Gain6/1 -> N_d/1  "n_d"
  Gain1/1 -> Integrator1/1
  Integrator1/1 -> Gain3/1, Gain2/1  "i_a"
  Integrator2/1 -> Omega_d/1, Gain6/1, Gain/1  "Omega_d"
  Gain4/1 -> Ускорени/1, Integrator2/1
  Sum/1 -> Gain1/1
  Gain2/1 -> Sum/3
  Gain7/1 -> Sum1/2
  Gain/1 -> Sum/1
  Sum1/1 -> Gain4/1

== system sim2/Subsystem/МПЛ/Subsystem ==
  M_h : Inport
  U : Inport  Port=2
  Gain : Gain  Gain=U_nom/w_0
  Gain1 : Gain  Gain=1/L_a
  Gain2 : Gain  Gain=R_a
  Gain3 : Gain  Gain=k_m
  Gain4 : Gain  Gain=1/J_sum
  Gain6 : Gain  Gain=60/(2*pi)
  Gain7 : Gain
  Integrator1 : Integrator
  Integrator2 : Integrator
  Scope : Scope
      settings: ActiveDisplayYMinimum=-1  ActiveDisplayYMaximum=1
  Sum : Sum  Inputs=-+-
  Sum1 : Sum  Inputs=|+-
  N_d : Outport
  Omega_d : Outport  Port=2
  Ускорени : Outport  Port=3
  wires:
  U/1 -> Sum/2
  Gain3/1 -> Sum1/1  "M"
  M_h/1 -> Scope/1, Gain7/1
  Gain6/1 -> N_d/1  "n_d"
  Gain1/1 -> Integrator1/1
  Integrator1/1 -> Gain3/1, Gain2/1  "i_a"
  Integrator2/1 -> Omega_d/1, Gain6/1, Gain/1  "Omega_d"
  Gain4/1 -> Ускорени/1, Integrator2/1
  Sum/1 -> Gain1/1
  Gain2/1 -> Sum/3
  Gain7/1 -> Sum1/2
  Gain/1 -> Sum/1
  Sum1/1 -> Gain4/1

== system sim2/Subsystem/МПП/Subsystem ==
  M_h : Inport
  U : Inport  Port=2
  Gain : Gain  Gain=U_nom/w_0
  Gain1 : Gain  Gain=1/L_a
  Gain2 : Gain  Gain=R_a
  Gain3 : Gain  Gain=k_m
  Gain4 : Gain  Gain=1/J_sum
  Gain6 : Gain  Gain=60/(2*pi)
  Gain7 : Gain
  Integrator1 : Integrator
  Integrator2 : Integrator
  Scope : Scope
      settings: ActiveDisplayYMinimum=-1  ActiveDisplayYMaximum=1
  Sum : Sum  Inputs=-+-
  Sum1 : Sum  Inputs=|+-
  N_d : Outport
  Omega_d : Outport  Port=2
  Ускорени : Outport  Port=3
  wires:
  U/1 -> Sum/2
  Gain3/1 -> Sum1/1  "M"
  M_h/1 -> Scope/1, Gain7/1
  Gain6/1 -> N_d/1  "n_d"
  Gain1/1 -> Integrator1/1
  Integrator1/1 -> Gain3/1, Gain2/1  "i_a"
  Integrator2/1 -> Omega_d/1, Gain6/1, Gain/1  "Omega_d"
  Gain4/1 -> Ускорени/1, Integrator2/1
  Sum/1 -> Gain1/1
  Gain2/1 -> Sum/3
  Gain7/1 -> Sum1/2
  Gain/1 -> Sum/1
  Sum1/1 -> Gain4/1
